simulink model "Router_communication"  (R2025a)
settings: Solver=VariableStepAuto  StartTime=0.0  StopTime=30  RelTol=1e-3
InitFcn:
  | %% Simulation parameters and waypoint trajectory
  | % Initial drone positions.
  | init_0=[0;0;0];
  | d_s=4;
  | init_1=init_0+d_s*[-1.1;0.1;0];
  | init_2=init_0+d_s*[0.3;-1.5;0];
  | init_3=init_0+d_s*[0.2;1.8;0];
  | init_4=init_0+d_s*[1.6;0.4;0];
  | 
  | Threshold = 1000*ones(45,1);
  | for i=1:9:37
  |     Threshold(i:i+2)=10;
  | end
  | gain_2=1;
  | 
  | % Router queues and background traffic.
  | router_buffer=5;
  | router_bandwith=20;
  | router_init_queue=3;
  | traffic_mean=20;
  | traffic_variance=1;
  | 
  | 
  | % Desired formation offsets.
  | init_f_0=[0;0;0];
  | d_f=1;
  | init_f_1=init_0+d_f*[-1;0;0];
  | init_f_2=init_0+d_f*[0;-1;0];
  | init_f_3=init_0+d_f*[0;1;0];
  | init_f_4=init_0+d_f*[1;0;0];
  | 
  | % Quadrotor mass and inertia.
  | mass = 1.2;
  | Ib   = diag([1.2416 1.2416 2*1.2416]);
  | 
  | % Time grid and waypoint trajectory.
  | Ts        = 0.001;
  | ttot      = 20;
  | tdead     = 10;
  | totalTime = ttot + tdead;
  | Nsamples  = 3000;
  | t_sample  = linspace(0, totalTime, Nsamples);
  | t=t_sample;
  | waypoints = [ ...
  |              0  0 -2 0;
  |              3  4 -5 0;
  |              2  1 -8 0;
  |              0 0 -10 0];
  | 
  | M    = size(waypoints,1);
  | t_wp = linspace(0, ttot, M);
  | 
  | p_d      = zeros(4, Nsamples);
  | dot_p_d  = zeros(4, Nsamples);
  | ddot_p_d = zeros(4, Nsamples);
  | 
  | idx_traj = t_sample <= ttot;
  | t_active = t_sample(idx_traj);
  | 
  | % Build position and yaw splines with zero endpoint velocities.
  | ... (+28 lines)
undefined symbols (not defined in the file): A_diacenza, K
libraries: robotcorelib x5, dspsigops x1, uavutilslib x1
(part 3 of 3)

== matlab function Router_communication/MATLAB Function2 ==
  data: M input; vec output; V input; A input
function vec = concatena_colonne(M, V, A)
% Stack state columns for the network controller.
    C = zeros(3, 15);

    C(:, 1:3:end) = M;
    C(:, 2:3:end) = V;
    C(:, 3:3:end) = A;

    vec = C(:);
end

== matlab function Router_communication/Subsystem1/Subsystem_1/Inner-loop control/Inner-loop control ==
  data: Rb_des output size=[3,3]; omega_bb_des output size=3; tau output size=3; zb_des input size=3; Rb input size=[3,3]; dot_Rb_des input size=[3,3]; omega_bb input size=3; dot_omega_bb_des input size=3; xb_des input size=3; Ib parameter size=[3,3]; err_R output size=3; err_W output size=3
function [Rb_des,omega_bb_des,tau,err_R,err_W] = fcn(zb_des,Rb,dot_Rb_des,omega_bb,dot_omega_bb_des,xb_des,Ib)
% Geometric attitude control from rotation and angular-velocity errors.


k_rx = 50;
k_ry = 50;
k_rz = 50;

k_wx = 50;
k_wy = 50;
k_wz = 50;

K_r = diag([k_rx, k_ry, k_rz]);
K_w = diag([k_wx, k_wy, k_wz]);


% Construct the desired rotation matrix from the requested body axes.
yb_des = (skew(zb_des)*xb_des)/norm(skew(zb_des)*xb_des);

Rb_des = [skew(yb_des)*zb_des, yb_des, zb_des];

omega_bb_des = wedge(Rb_des&apos;*dot_Rb_des);

err_R = 0.5*wedge(Rb_des&apos;*Rb - Rb&apos;*Rb_des);

err_W = omega_bb - Rb&apos;*Rb_des*omega_bb_des;

% Combine attitude feedback with rigid-body compensation.
tau = -K_r*err_R - K_w*err_W + skew(omega_bb)*Ib*omega_bb - Ib*(skew(omega_bb)*Rb&apos;*Rb_des*omega_bb_des-Rb&apos;*Rb_des*dot_omega_bb_des); 

end

function S = skew(v)
% Matrix representation of the cross product.
if(numel(v)~= 1)
S= [0 -v(3) v(2); 
    v(3) 0 -v(1);
    -v(2) v(1) 0];
else
S= zeros(3);
end
end

function v = wedge(S)
% Extract the vector associated with a skew-symmetric matrix.
v1 = S(3,2);
v2 = S(1,3);
v3 = S(2,1);
v = [v1 v2 v3]&apos;;
end
